simulink model "robot_ver2_multibody"  (R2024b)
settings: Solver=ode15s  StartTime=0.0  StopTime=8  MaxStep=.01  RelTol=1e-6  AbsTol=1e-8
PostLoadFcn:
  | addpath(fullfile(fileparts(get_param(bdroot,'FileName')), '..','CAD','URDF_Assembly_Robot_ver2','meshes'));
InitFcn:
  | addpath(fullfile(fileparts(get_param(bdroot,'FileName')), '..','CAD','URDF_Assembly_Robot_ver2','meshes'));
model workspace (MAT data in the model file):
  demoKd = [33.1365056218 98.6550272627 34.0147620615 3.49229083301 1.35827925784 0.348859210513]
  demoKp = [160 500 250 25 20 8]
  demoQ = [0 0.01 0.02 0.03 0.04 0.05 0.06 0.07 0.08 0.09 0.1 0.11 ... (5607 elements, 801x7)]
  demoQd = [0 0.01 0.02 0.03 0.04 0.05 0.06 0.07 0.08 0.09 0.1 0.11 ... (5607 elements, 801x7)]
  holdTorque = [-1.77561199876e-21 -27.0149765766 27.0149765766 -1.68106782493 1.17384936667e-14 0.0935435424716]
  initialQ = [0 0 0 0 0 0]
  multibodyInfo.robotID = 'robot_ver2'
  multibodyInfo.schemaVersion = 1
  multibodyInfo.urdfSHA256 = '4375e6be56b72db950ac87d5631842c692121a0d0489fcb89f928996cc18049b'
  multibodyInfo.jointNames = ["Joint_1" "Joint_2" "Joint_3" "Joint_4" "Joint_5" "Joint_6"]
  multibodyInfo.gravity = [0 0 -9.81]
  multibodyInfo.units.torque = 'N m'
  multibodyInfo.units.position = 'rad'
  multibodyInfo.units.velocity = 'rad/s'
  multibodyInfo.units.acceleration = 'rad/s^2'
  multibodyInfo.source = 'robots/robot_ver2/CAD/URDF_Assembly_Robot_ver2/urdf/URDF_Assembly_Robot_ver2.urdf'
  multibodyInfo.builtAt = '2026-10-29 07:24:52'
  multibodyInfo.demoOnly = 1
  multibodyInfo.motorRatingsIncluded = 0
  multibodyInfo.contactsIncluded = 0
undefined symbols (not defined in the file or in its folder): X, Y, Z
libraries: sm_lib x67, nesl_utility x27
(part 1 of 3)
settings Model: Creator=pc  LastModifiedBy=pc

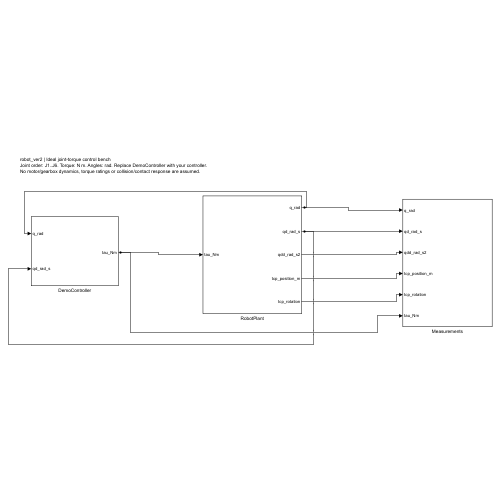
[thumbnail: Simulink's stored preview of the top-level diagram]
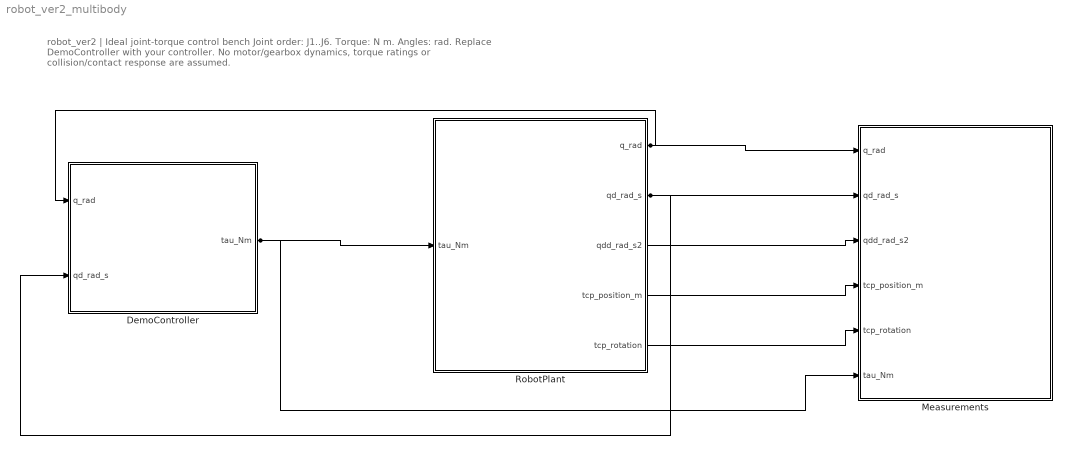
== system robot_ver2_multibody ==
  note: robot_ver2 | Ideal joint-torque control bench
      | Joint order: J1..J6. Torque: N m. Angles: rad. Replace DemoController with your controller.
      | No motor/gearbox dynamics, torque ratings or collision/contact response are assumed.
  DemoController : Subsystem
  Measurements : Subsystem
  RobotPlant : Subsystem
  wires:
  DemoController/1(tau_Nm) -> RobotPlant/1(tau_Nm), Measurements/6(tau_Nm)
  RobotPlant/1(q_rad) -> DemoController/1(q_rad), Measurements/1(q_rad)
  RobotPlant/2(qd_rad_s) -> DemoController/2(qd_rad_s), Measurements/2(qd_rad_s)
  RobotPlant/3(qdd_rad_s2) -> Measurements/3(qdd_rad_s2)
  RobotPlant/4(tcp_position_m) -> Measurements/4(tcp_position_m)
  RobotPlant/5(tcp_rotation) -> Measurements/5(tcp_rotation)
